simulink model "Vehicle_Drive"  (R2026a)
settings: Solver=FixedStepAuto  StopTime=10  FixedStep=.001  EnableMultiTasking=on
InitFcn:
  | addpath('C:\Users\jpgre\OneDrive\Documents\ChatGPT\ETE 4851 Project\outputs\ina219_diagnostic','C:\Users\jpgre\OneDrive\Documents\ChatGPT\ETE 4851 Project\outputs\motor_imu');
libraries: stm32f4xxblockslib x4, stm32blockslib x4
settings Model: STM32="{\"DigitalPortWrite\":[{\"ID\":\"92\"},{\"ID\":\"93\"},{\"ID\":\"116\"}],\"PWMOutput\":{\"ID\":\"91\"},\"UARTWrite\":[{\"ID\":\"103\"},{\"ID\":\"110\"}],\"UARTRead\":[{\"ID\":\"98\"},{\"ID\":\"117\"}]}"  SimulationMode=external  ExtModeTrigDuration=10  Creator=smboskovich  LastModifiedBy=jpgre
settings OptimizationCC: PassReuseOutputArgsThreshold=0.0  MaxStackSize=512
settings HardwareCC: ProdLargestAtomicInteger=Long  ProdLargestAtomicFloat=Double  ProdHWDeviceType=ARM Compatible->ARM Cortex-M
settings RTWCC: SystemTargetFile=ert.tlc  HardwareBoard=STM32F7xx Based (Double precision FPU)  TLCOptions=-aInlineSetEventsForThisBaseRateFcn=TLC_FALSE -aSuppressMultiTaskScheduler=TLC_FALSE -aRateBasedStepFcn=1  GenerateReport=on  CustomInclude=.  CustomSource=vehicle_io.c current_ina219.c  Toolchain=GNU Tools for STM32  BuildConfiguration=Faster Runs  LaunchReport=on  Description=Embedded Coder
settings ERTTargetCC: ExtModeTransport=3.0  ExtModeStaticAllocSize=2048.0  DynamicArrayContainerType=coder::array  CodeReplacementLibrary=ARM Cortex-M  ERTCustomFileBanners=off  SupportContinuousTime=on  SupportNonInlinedSFcns=on  ModelStepFunctionPrototypeControlCompliant=off

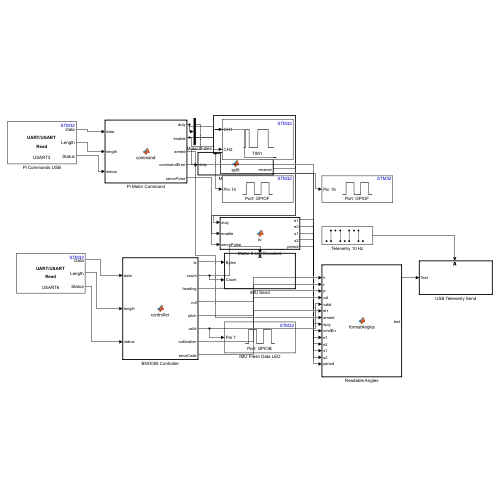
[thumbnail: Simulink's stored preview of the top-level diagram]
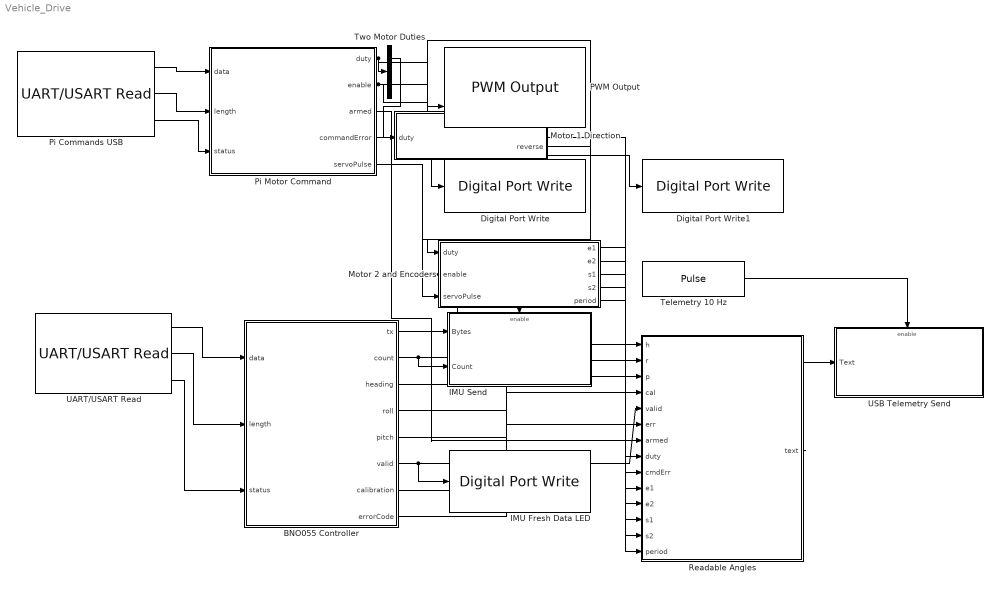
== system Vehicle_Drive ==
  BNO055 Controller : MATLAB Function  TreatAsAtomicUnit=on
  Digital Port Write : stm32f4xxblockslib/Digital Port Write  PortName=GPIOF  PinNumber=[14]  ReadOperation=off  IOAsArray=off  EnableSimPort=off  hoistedMaskSrc=ECSoC/ECSimCodegen/Digital Port Write
      settings: LibrarySourceBlock=stm32h7xxblockslib/Digital Port Write
  Digital Port Write1 : stm32f4xxblockslib/Digital Port Write  PortName=GPIOF  PinNumber=[15]  ReadOperation=off  IOAsArray=off  EnableSimPort=off  hoistedMaskSrc=ECSoC/ECSimCodegen/Digital Port Write
      settings: LibrarySourceBlock=stm32h7xxblockslib/Digital Port Write
  IMU Fresh Data LED : stm32f4xxblockslib/Digital Port Write  PortName=GPIOB  PinNumber=7  ReadOperation=off  IOAsArray=off  EnableSimPort=off  hoistedMaskSrc=ECSoC/ECSimCodegen/Digital Port Write
      settings: LibrarySourceBlock=stm32h7xxblockslib/Digital Port Write
  IMU Send : Subsystem
  Motor 1 Direction : MATLAB Function  TreatAsAtomicUnit=on
  Motor 2 and Encoders : MATLAB Function  TreatAsAtomicUnit=on
  PWM Output : stm32f4xxblockslib/PWM Output  ProcessorFamily=STM32G4  TimerModule=TIM1  DutycycleUnits=Percentage  EnableChannel1=on  EnableCaptureCompare1Input=off  EnableCaptureCompare1ComplementaryInput=off  EnableOutputCompare1ModeInput=off  EnableChannel2=on  EnableCaptureCompare2Input=off  EnableCaptureCompare2ComplementaryInput=off  EnableOutputCompare2ModeInput=off  EnableChannel3=off  EnableCaptureCompare3Input=off  EnableCaptureCompare3ComplementaryInput=off  EnableOutputCompare3ModeInput=off  EnableChannel4=off  EnableCaptureCompare4Input=off  EnableCaptureCompare4ComplementaryInput=off  EnableOutputCompare4ModeInput=off  EnableChannel5=off  EnableCaptureCompare5Input=off  EnableOutputCompare5ModeInput=off  EnableChannel6=off  EnableCaptureCompare6Input=off  EnableOutputCompare6ModeInput=off  EnableCounterInput=off  EnableMainOutputInput=off  EnableFrequencyInput=off  SetRCAfterCE=off  OutputDirection=off  OutputMainOutputEnableStatus=off  SampleTime=0.001  EnableSimPort=off  EnableUpdateEvent=off  EnableCaptureCompare1Event=off  EnableCaptureCompare2Event=off  EnableCaptureCompare3Event=off  EnableCaptureCompare4Event=off  EnableTriggerEvent=off  EnableBreakEvent=off  EnableBreakEvent2=off  hoistedMaskSrc=ECSoC/ECSimCodegen/PWM Output
      settings: LibrarySourceBlock=stm32h7xxblockslib/PWM Output
  Pi Commands USB : stm32blockslib/UART//USART Read  UARTModule=USART3  DataType=uint8  DataLength=1  BlockingMode=off  BlockingTimeout=0.1  OutputLength=on  OutputStatus=on  SampleTime=0.001
  Pi Motor Command : MATLAB Function  TreatAsAtomicUnit=on
  Readable Angles : MATLAB Function  TreatAsAtomicUnit=on
  Telemetry 10 Hz : DiscretePulseGenerator  Period=100  SampleTime=0.001
  Two Motor Duties : Demux  Outputs=2
  UART/USART Read : stm32blockslib/UART//USART Read  UARTModule=USART6  DataType=uint8  DataLength=1  BlockingMode=off  BlockingTimeout=0.1  OutputLength=on  OutputStatus=on  SampleTime=0.001
  USB Telemetry Send : Subsystem
  wires:
  UART/USART Read/1 -> BNO055 Controller/1(data)
  UART/USART Read/2 -> BNO055 Controller/2(length)
  UART/USART Read/3 -> BNO055 Controller/3(status)
  BNO055 Controller/1(tx) -> IMU Send/1(Bytes)
  BNO055 Controller/2(count) -> IMU Send/2(Count), IMU Send/Enable
  BNO055 Controller/3(heading) -> Readable Angles/1(h)
  BNO055 Controller/4(roll) -> Readable Angles/2(r)
  BNO055 Controller/5(pitch) -> Readable Angles/3(p)
  BNO055 Controller/7(calibration) -> Readable Angles/4(cal)
  BNO055 Controller/6(valid) -> Readable Angles/5(valid), IMU Fresh Data LED/1
  BNO055 Controller/8(errorCode) -> Readable Angles/6(err)
  Readable Angles/1(text) -> USB Telemetry Send/1(Text)
  Telemetry 10 Hz/1 -> USB Telemetry Send/Enable
  Pi Commands USB/1 -> Pi Motor Command/1(data)
  Pi Commands USB/2 -> Pi Motor Command/2(length)
  Pi Commands USB/3 -> Pi Motor Command/3(status)
  Pi Motor Command/1(duty) -> Readable Angles/8(duty), Two Motor Duties/1
  Pi Motor Command/2(enable) -> Digital Port Write/1, Digital Port Write1/1, Motor 2 and Encoders/2(enable)
  Pi Motor Command/3(armed) -> Readable Angles/7(armed)
  Pi Motor Command/4(commandError) -> Readable Angles/9(cmdErr)
  Two Motor Duties/1 -> Motor 1 Direction/1(duty)
  Motor 1 Direction/1(forward) -> PWM Output/1
  Motor 1 Direction/2(reverse) -> PWM Output/2
  Two Motor Duties/2 -> Motor 2 and Encoders/1(duty)
  Pi Motor Command/5(servoPulse) -> Motor 2 and Encoders/3(servoPulse)
  Motor 2 and Encoders/1(e1) -> Readable Angles/10(e1)
  Motor 2 and Encoders/2(e2) -> Readable Angles/11(e2)
  Motor 2 and Encoders/3(s1) -> Readable Angles/12(s1)
  Motor 2 and Encoders/4(s2) -> Readable Angles/13(s2)
  Motor 2 and Encoders/5(period) -> Readable Angles/14(period)

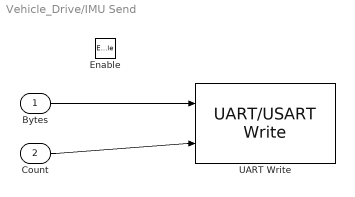
== system Vehicle_Drive/IMU Send ==
  Bytes : Inport
  Count : Inport  Port=2
  Enable : EnablePort
  UART Write : stm32blockslib/UART//USART Write  UARTModule=USART6  LengthOfDataToSend=on  BlockingMode=off  BlockingTimeout=0.1  OutputStatus=off
  wires:
  Bytes/1 -> UART Write/1
  Count/1 -> UART Write/2

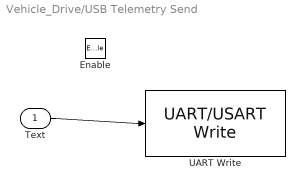
== system Vehicle_Drive/USB Telemetry Send ==
  Text : Inport
  Enable : EnablePort
  UART Write : stm32blockslib/UART//USART Write  UARTModule=USART3  LengthOfDataToSend=off  BlockingMode=off  BlockingTimeout=0.1  OutputStatus=off
  wires:
  Text/1 -> UART Write/1

== matlab function Vehicle_Drive/Readable Angles ==
  data: h input; text output; r input; p input; cal input; valid input; err input; armed input; duty input; cmdErr input; e1 input; e2 input; s1 input; s2 input; period input
function text = formatAngles(h,r,p,cal,valid,err,armed,duty,cmdErr,e1,e2,s1,s2,period)
text=vehicle_text(h,r,p,cal,valid,err,armed,duty,cmdErr,e1,e2,s1,s2,period);
end

== matlab function Vehicle_Drive/BNO055 Controller ==
  data: data input; tx output; length input; status input; count output; heading output; roll output; pitch output; valid output; calibration output; errorCode output
function [tx,count,heading,roll,pitch,valid,calibration,errorCode] = controller(data,length,status)
[tx,count,heading,roll,pitch,valid,calibration,errorCode] = bno055_controller(data,length,status);
end

== matlab function Vehicle_Drive/Pi Motor Command ==
  data: data input; duty output; length input; status input; enable output; armed output; commandError output; servoPulse output
function [duty,enable,armed,commandError,servoPulse] = command(data,length,status)
[duty,enable,armed,commandError,servoPulse] = vehicle_command(data,length,status);
end

== matlab function Vehicle_Drive/Motor 1 Direction ==
  data: duty input; forward output; reverse output
function [forward,reverse]=split(duty)
forward=max(0,duty); reverse=max(0,-duty);
end

== matlab function Vehicle_Drive/Motor 2 and Encoders ==
  data: duty input; e1 output; enable input; servoPulse input; e2 output; s1 output; s2 output; period output
function [e1,e2,s1,s2,period] = io(duty,enable,servoPulse)
%#codegen
e1=uint16(0); e2=uint16(0); s1=uint16(0); s2=uint16(0); period=uint16(0);
if ~coder.target('MATLAB') && ~coder.target('Sfun')
coder.cinclude('vehicle_io.h');
coder.ceval('vehicle_io',double(duty),uint8(enable),coder.wref(e1),coder.wref(e2));
coder.ceval('vehicle_servo_io',double(servoPulse(1)),double(servoPulse(2)));
coder.ceval('vehicle_servo_status',coder.wref(s1),coder.wref(s2),coder.wref(period));
end
end
